simulink model "TP1_commande_des_retroviseurs_Simulink"  (R2022b)
settings: Solver=VariableStepAuto  StartTime=0.0  StopTime=inf  RelTol=1e-3
libraries: simulink x8
settings Model: Creator=HP  LastModifiedBy=HP

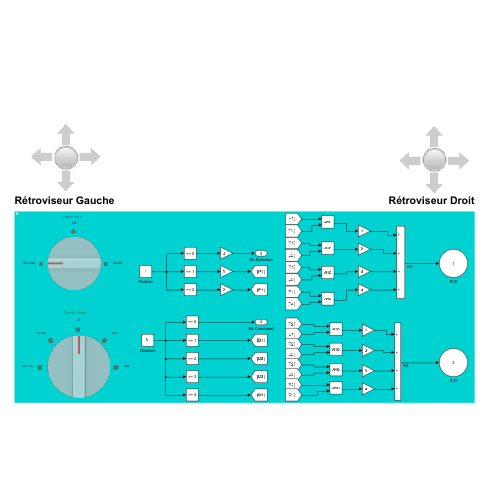
[thumbnail: Simulink's stored preview of the top-level diagram]
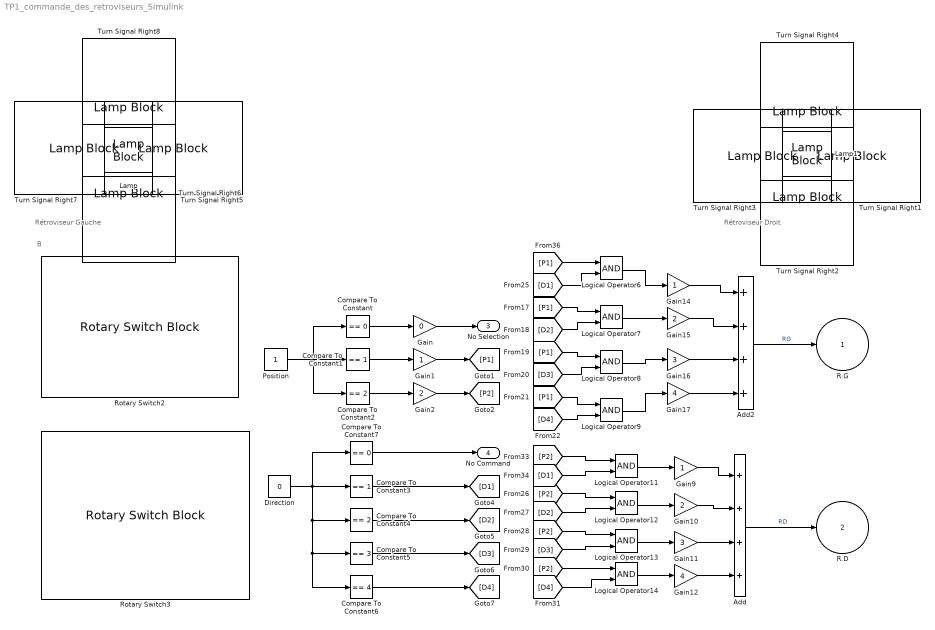
== system TP1_commande_des_retroviseurs_Simulink ==
  note: B
  note: Rétroviseur Droit
  note: Rétroviseur Gauche
  Add : Sum  Inputs=++++
  Add2 : Sum  Inputs=++++
  Compare To Constant : simulink/Logic and Bit Operations/Compare To Constant  relop===  const=0  OutDataTypeStr=boolean
  Compare To Constant1 : simulink/Logic and Bit Operations/Compare To Constant  relop===  const=1  OutDataTypeStr=boolean
  Compare To Constant2 : simulink/Logic and Bit Operations/Compare To Constant  relop===  const=2  OutDataTypeStr=boolean
  Compare To Constant3 : simulink/Logic and Bit Operations/Compare To Constant  relop===  const=1  OutDataTypeStr=boolean
  Compare To Constant4 : simulink/Logic and Bit Operations/Compare To Constant  relop===  const=2  OutDataTypeStr=boolean
  Compare To Constant5 : simulink/Logic and Bit Operations/Compare To Constant  relop===  const=3  OutDataTypeStr=boolean
  Compare To Constant6 : simulink/Logic and Bit Operations/Compare To Constant  relop===  const=4  OutDataTypeStr=boolean
  Compare To Constant7 : simulink/Logic and Bit Operations/Compare To Constant  relop===  const=0  OutDataTypeStr=boolean
  Direction : Constant  Value=0
  Gain : Gain  Gain=0
  Gain1 : Gain
  Gain10 : Gain  Gain=2
  Gain11 : Gain  Gain=3
  Gain12 : Gain  Gain=4
  Gain14 : Gain
  Gain15 : Gain  Gain=2
  Gain16 : Gain  Gain=3
  Gain17 : Gain  Gain=4
  Gain2 : Gain  Gain=2
  Gain9 : Gain
  Lamp : LampBlock  LabelPosition=Hide
  Lamp1 : LampBlock  LabelPosition=Hide
  Logical Operator{6..9,11..14} (8 alike) : Logic  AllPortsSameDT=off  OutDataTypeStr=boolean
  Position : Constant
  Rotary Switch2 : RotarySwitchBlock
      settings: Values={{'Gauche', 'Off', 'Droite'}, [1 0 2]}
  Rotary Switch3 : RotarySwitchBlock
      settings: Values={{'Gauche', 'Droite', 'Off', 'Haut', 'Bas'}, [1 2 0 3 4]}
  Turn Signal Right{1..8} (8 alike) : LampBlock  LabelPosition=Hide  Icon=TurnSignalRight
  R.G : Outport
  R.D : Outport  Port=2
  No Selection : Outport  Port=3
  No Command : Outport  Port=4
  wires:
  Position/1 -> Compare To Constant/1, Compare To Constant2/1, Compare To Constant1/1
  Compare To Constant2/1 -> Gain2/1
  Compare To Constant/1 -> Gain/1
  Compare To Constant1/1 -> Gain1/1
  Direction/1 -> Compare To Constant5/1, Compare To Constant6/1, Compare To Constant4/1, Compare To Constant7/1, Compare To Constant3/1
  Gain/1 -> No Selection/1
  Gain1/1 -> [P1]
  Gain2/1 -> [P2]
  Compare To Constant5/1 -> [D3]
  Compare To Constant6/1 -> [D4]
  Compare To Constant4/1 -> [D2]
  Compare To Constant3/1 -> [D1]
  Compare To Constant7/1 -> No Command/1
  [D4] -> Logical Operator14/2
  [P2] -> Logical Operator14/1
  [D3] -> Logical Operator13/2
  [P2] -> Logical Operator13/1
  [D2] -> Logical Operator12/2
  [P2] -> Logical Operator12/1
  [D1] -> Logical Operator11/2
  [P2] -> Logical Operator11/1
  Logical Operator11/1 -> Gain9/1
  Logical Operator12/1 -> Gain10/1
  Logical Operator13/1 -> Gain11/1
  Logical Operator14/1 -> Gain12/1
  Logical Operator9/1 -> Gain17/1
  Logical Operator8/1 -> Gain16/1
  Logical Operator7/1 -> Gain15/1
  Logical Operator6/1 -> Gain14/1
  [P1] -> Logical Operator6/1
  [D1] -> Logical Operator6/2
  [P1] -> Logical Operator7/1
  [D2] -> Logical Operator7/2
  [P1] -> Logical Operator8/1
  [D3] -> Logical Operator8/2
  [P1] -> Logical Operator9/1
  [D4] -> Logical Operator9/2
  Gain9/1 -> Add/1
  Gain10/1 -> Add/2
  Gain11/1 -> Add/3
  Gain12/1 -> Add/4
  Gain14/1 -> Add2/1
  Gain15/1 -> Add2/2
  Gain16/1 -> Add2/3
  Gain17/1 -> Add2/4
  Add2/1 -> R.G/1  "RG"
  Add/1 -> R.D/1  "RD"
